simulink model "phase3_scheduler_application"  (R2026a)
settings: Solver=FixedStepDiscrete  EnableMultiTasking=on
settings Model: Creator=The MathWorks, Inc.  LastModifiedBy=rayyu
settings SolverCC: PositivePriorityOrder=on
settings HardwareCC: ProdBitPerLong=64.0  ProdLargestAtomicInteger=LongLong  ProdLargestAtomicFloat=Double  ProdHWDeviceType=ARM Compatible->ARM Cortex-A (64-bit)  HardwareBoardFeatureSet=SoCBlockset
settings RTWCC: SystemTargetFile=ert.tlc  HardwareBoard=Xilinx Zynq UltraScale+ MPSoC ZCU102 Evaluation Kit  TLCOptions="-aInlineSetEventsForThisBaseRateFcn=TLC_FALSE -aSuppressMultiTaskScheduler=TLC_FALSE  -aRateBasedStepFcn=0"  GenerateReport=on  Toolchain=Linaro AArch64 Linux v6.3.1  IncludeHyperlinkInReport=on  LaunchReport=on  GenerateTraceInfo=on  GenerateTraceReport=on  GenerateTraceReportSl=on  GenerateTraceReportSf=on  GenerateTraceReportEml=on  Description=Embedded Coder
settings ERTTargetCC: ExtModeTransport=2.0  DynamicArrayContainerType=coder::array

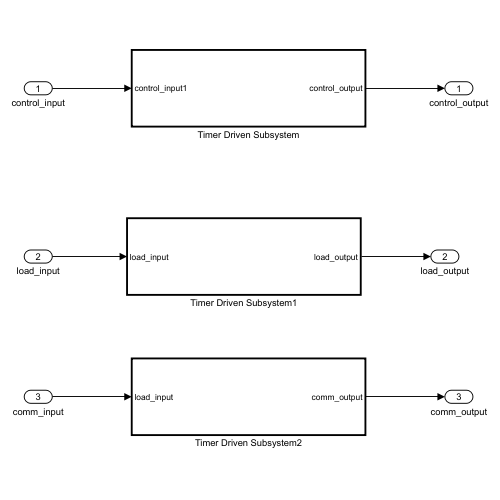
[thumbnail: Simulink's stored preview of the top-level diagram]
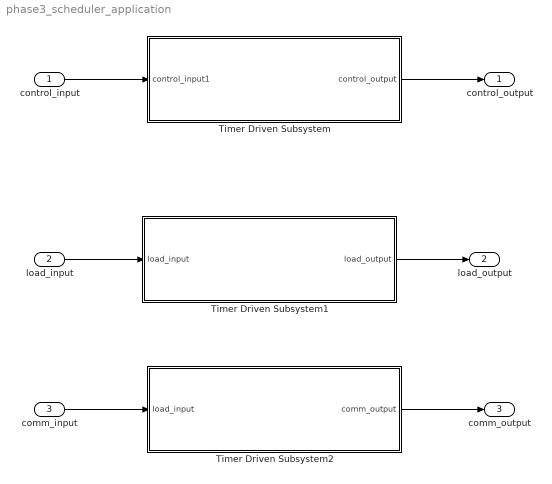
== system phase3_scheduler_application ==
  control_input : Inport
  load_input : Inport  Port=2
  comm_input : Inport  Port=3
  Timer Driven Subsystem : Subsystem  TreatAsAtomicUnit=on
  Timer Driven Subsystem1 : Subsystem  TreatAsAtomicUnit=on
  Timer Driven Subsystem2 : Subsystem  TreatAsAtomicUnit=on
  control_output : Outport  VectorParamsAs1DForOutWhenUnconnected=off
  load_output : Outport  Port=2  VectorParamsAs1DForOutWhenUnconnected=off
  comm_output : Outport  Port=3
  wires:
  Timer Driven Subsystem/1(control_output) -> control_output/1
  control_input/1 -> Timer Driven Subsystem/1(control_input1)
  load_input/1 -> Timer Driven Subsystem1/1(load_input)
  Timer Driven Subsystem1/1(load_output) -> load_output/1
  comm_input/1 -> Timer Driven Subsystem2/1(load_input)
  Timer Driven Subsystem2/1(comm_output) -> comm_output/1

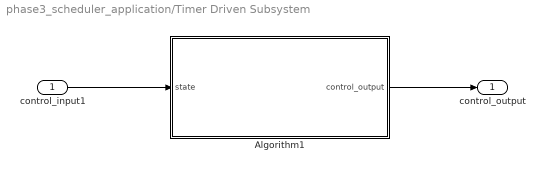
== system phase3_scheduler_application/Timer Driven Subsystem ==
  control_input1 : Inport  SampleTime=0.01
  Algorithm1 : Subsystem
  control_output : Outport  VectorParamsAs1DForOutWhenUnconnected=off
  wires:
  Algorithm1/1(control_output) -> control_output/1
  control_input1/1 -> Algorithm1/1(state)

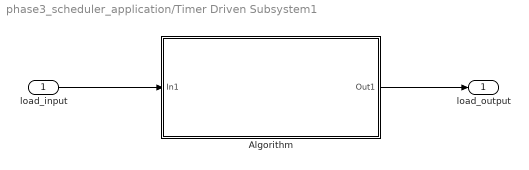
== system phase3_scheduler_application/Timer Driven Subsystem1 ==
  load_input : Inport  SampleTime=0.05
  Algorithm : Subsystem
  load_output : Outport  VectorParamsAs1DForOutWhenUnconnected=off
  wires:
  Algorithm/1(Out1) -> load_output/1
  load_input/1 -> Algorithm/1(In1)

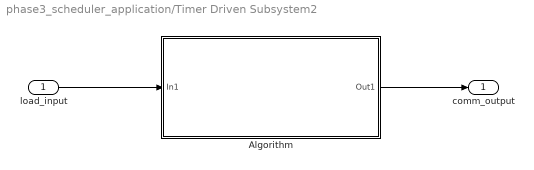
== system phase3_scheduler_application/Timer Driven Subsystem2 ==
  load_input : Inport  SampleTime=0.005
  Algorithm : Subsystem
  comm_output : Outport  VectorParamsAs1DForOutWhenUnconnected=off
  wires:
  load_input/1 -> Algorithm/1(In1)
  Algorithm/1(Out1) -> comm_output/1

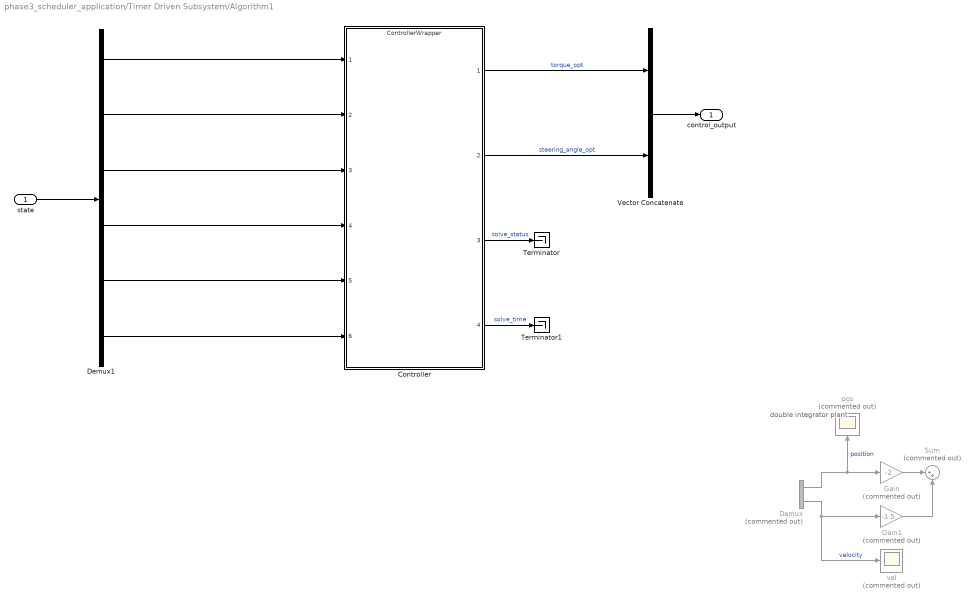
== system phase3_scheduler_application/Timer Driven Subsystem/Algorithm1 ==
  note: double integrator plant
  state : Inport
  Controller : ModelReference  ModelNameDialog=ControllerWrapper.slx  SimulationMode=Normal  ModelReferenceVersion=1.41
  Demux : Demux  Commented=on  Outputs=2
  Demux1 : Demux  Outputs=6
  Gain : Gain  Commented=on  Gain=-2
  Gain1 : Gain  Commented=on  Gain=-1.5
  Sum : Sum  Commented=on  Inputs=|++
  Terminator : Terminator
  Terminator1 : Terminator
  Vector Concatenate : Concatenate
  pos : Scope  Commented=on
      settings: ActiveDisplayYMinimum=0.97933239858184118  ActiveDisplayYMaximum=1.0022964001575732
  vel : Scope  Commented=on
      settings: ActiveDisplayYMinimum=-0.28436863626504516  ActiveDisplayYMaximum=0.031596515140560569
  control_output : Outport
  wires:
  Gain/1 -> Sum/1
  state/1 -> Demux1/1
  Demux/1 -> Gain/1, pos/1  "position"
  Demux/2 -> Gain1/1, vel/1  "velocity"
  Gain1/1 -> Sum/2
  Demux1/1 -> Controller/1
  Demux1/2 -> Controller/2
  Demux1/3 -> Controller/3
  Demux1/4 -> Controller/4
  Demux1/5 -> Controller/5
  Demux1/6 -> Controller/6
  Controller/1 -> Vector Concatenate/1  "torque_opt"
  Controller/2 -> Vector Concatenate/2  "steering_angle_opt"
  Controller/3 -> Terminator/1  "solve_status"
  Controller/4 -> Terminator1/1  "solve_time"
  Vector Concatenate/1 -> control_output/1

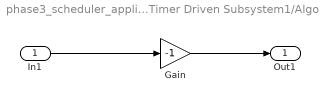
== system phase3_scheduler_application/Timer Driven Subsystem1/Algorithm ==
  In1 : Inport
  Gain : Gain  Gain=-1
  Out1 : Outport  VectorParamsAs1DForOutWhenUnconnected=off
  wires:
  In1/1 -> Gain/1
  Gain/1 -> Out1/1

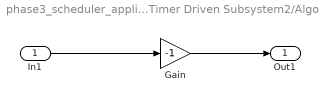
== system phase3_scheduler_application/Timer Driven Subsystem2/Algorithm ==
  In1 : Inport
  Gain : Gain  Gain=-1
  Out1 : Outport  VectorParamsAs1DForOutWhenUnconnected=off
  wires:
  Gain/1 -> Out1/1
  In1/1 -> Gain/1
